simulink model "all_afc_0001_0365"  (R2026a)
settings: Solver=ode15s  StopTime=simTime  FixedStep=5e-05  RelTol=1e-06  AbsTol=1e-06
undefined symbols (not defined in the file): AF_sensor_tol, fault_time, fuel_inj_tol, MAF_sensor_tol, measureTime, simTime, spec_num
(part 3 of 3)

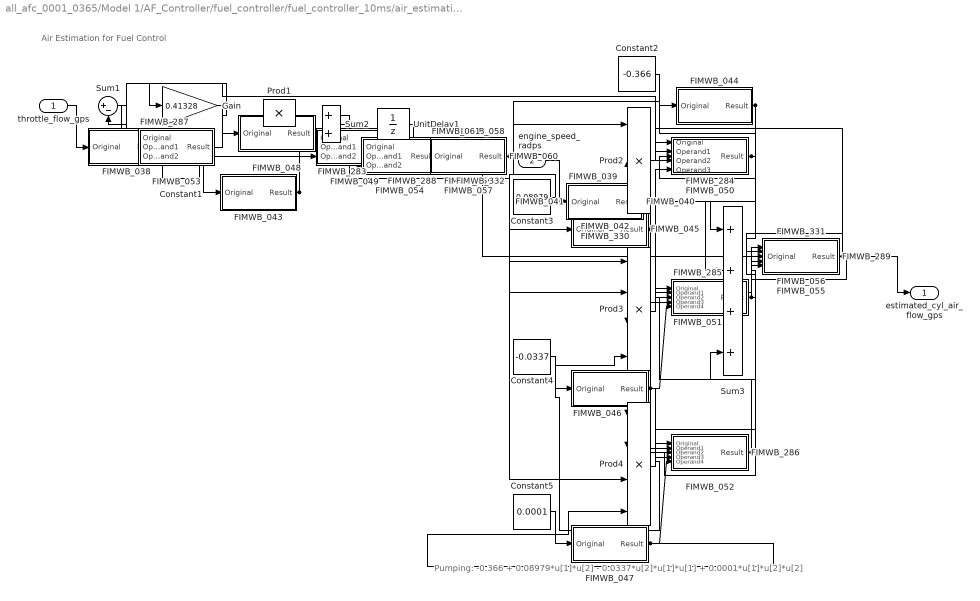
== system all_afc_0001_0365/Model 1/AF_Controller/fuel_controller/fuel_controller_10ms/air_estimation ==
  note: Air Estimation for Fuel Control
  note: Pumping: -0.366 + 0.08979*u[1]*u[2] - 0.0337*u[2]*u[1]*u[1] + 0.0001*u[1]*u[2]*u[2]
  throttle_flow_gps : Inport
  engine_speed_radps : Inport  Port=2
  Constant1 : Constant  Value=0.01  OutDataTypeStr=single  SampleTime=-1
      settings: AttributesFormatString=Sample Time (s)
  Constant2 : Constant  Value=-0.366  OutDataTypeStr=single  SampleTime=-1
  Constant3 : Constant  Value=0.08979  OutDataTypeStr=single  SampleTime=-1
  Constant4 : Constant  Value=-0.0337  OutDataTypeStr=single  SampleTime=-1
  Constant5 : Constant  Value=0.0001  OutDataTypeStr=single  SampleTime=-1
  FIMWB_038 : Subsystem  Tag=fimwb.fault.38
  FIMWB_039 : Subsystem  Tag=fimwb.fault.39
  FIMWB_040 : Subsystem  Tag=fimwb.fault.40
  FIMWB_041 : Subsystem  Tag=fimwb.fault.41
  FIMWB_042 : Subsystem  Tag=fimwb.fault.42
  FIMWB_043 : Subsystem  Tag=fimwb.fault.43
  FIMWB_044 : Subsystem  Tag=fimwb.fault.44
  FIMWB_045 : Subsystem  Tag=fimwb.fault.45
  FIMWB_046 : Subsystem  Tag=fimwb.fault.46
  FIMWB_047 : Subsystem  Tag=fimwb.fault.47
  FIMWB_048 : Subsystem  Tag=fimwb.fault.48
  FIMWB_049 : Subsystem  Tag=fimwb.fault.49
  FIMWB_050 : Subsystem  Tag=fimwb.fault.50
  FIMWB_051 : Subsystem  Tag=fimwb.fault.51
  FIMWB_052 : Subsystem  Tag=fimwb.fault.52
  FIMWB_053 : Subsystem  Tag=fimwb.fault.53
  FIMWB_054 : Subsystem  Tag=fimwb.fault.54
  FIMWB_055 : Subsystem  Tag=fimwb.fault.55
  FIMWB_056 : Subsystem  Tag=fimwb.fault.56
  FIMWB_057 : Subsystem  Tag=fimwb.fault.57
  FIMWB_058 : Subsystem  Tag=fimwb.fault.58
  FIMWB_059 : Subsystem  Tag=fimwb.fault.59
  FIMWB_060 : Subsystem  Tag=fimwb.fault.60
  FIMWB_061 : Subsystem  Tag=fimwb.fault.61
  FIMWB_283 : Subsystem  Tag=fimwb.fault.283
  FIMWB_284 : Subsystem  Tag=fimwb.fault.284
  FIMWB_285 : Subsystem  Tag=fimwb.fault.285
  FIMWB_286 : Subsystem  Tag=fimwb.fault.286
  FIMWB_287 : Subsystem  Tag=fimwb.fault.287
  FIMWB_288 : Subsystem  Tag=fimwb.fault.288
  FIMWB_289 : Subsystem  Tag=fimwb.fault.289
  FIMWB_330 : Subsystem  Tag=fimwb.fault.330
  FIMWB_331 : Subsystem  Tag=fimwb.fault.331
  FIMWB_332 : Subsystem  Tag=fimwb.fault.332
  Gain : Gain  Gain=0.41328  ParamDataTypeStr=single  OutDataTypeStr=Inherit: Inherit via back propagation  RndMeth=Simplest  SaturateOnIntegerOverflow=on
      settings: AttributesFormatString=RT/Vm
  Prod1 : Product  OutDataTypeStr=Inherit: Inherit via back propagation  RndMeth=Simplest
  Prod2 : Product  Inputs=3  OutDataTypeStr=Inherit: Inherit via back propagation  RndMeth=Simplest
  Prod3 : Product  Inputs=4  OutDataTypeStr=Inherit: Inherit via back propagation  RndMeth=Simplest
  Prod4 : Product  Inputs=4  OutDataTypeStr=Inherit: Inherit via back propagation  RndMeth=Simplest
  Sum1 : Sum  Inputs=|+-  OutDataTypeStr=Inherit: Inherit via back propagation  InputSameDT=on  RndMeth=Simplest
  Sum2 : Sum  OutDataTypeStr=Inherit: Inherit via back propagation  InputSameDT=on  RndMeth=Simplest
  Sum3 : Sum  Inputs=++++  OutDataTypeStr=Inherit: Inherit via back propagation  InputSameDT=on  RndMeth=Simplest
  UnitDelay1 : UnitDelay  InitialCondition=0.982  SampleTime=-1
      settings: AttributesFormatString=p0 = %<InitialCondition> (bar)
  estimated_cyl_air_flow_gps : Outport  VectorParamsAs1DForOutWhenUnconnected=off
  wires:
  Prod1/1 -> FIMWB_283/1(Original)
  Prod2/1 -> FIMWB_284/1(Original)
  Prod3/1 -> FIMWB_285/1(Original)
  Prod4/1 -> FIMWB_286/1(Original)
  Sum1/1 -> FIMWB_287/1(Original)
  Sum2/1 -> FIMWB_288/1(Original)
  Sum3/1 -> FIMWB_289/1(Original)
  engine_speed_radps/1 -> FIMWB_330/1(Original)
  FIMWB_330/1(Result) -> FIMWB_039/1(Original), FIMWB_040/1(Original), FIMWB_041/1(Original), FIMWB_042/1(Original)
  FIMWB_289/1(Result) -> FIMWB_331/1(Original)
  FIMWB_331/1(Result) -> FIMWB_055/1(Original), FIMWB_056/1(Original)
  UnitDelay1/1 -> FIMWB_332/1(Original)
  FIMWB_332/1(Result) -> FIMWB_057/1(Original), FIMWB_058/1(Original), FIMWB_059/1(Original), FIMWB_060/1(Original), FIMWB_061/1(Original)
  throttle_flow_gps/1 -> FIMWB_038/1(Original)
  FIMWB_038/1(Result) -> Sum1/1, FIMWB_287/2(Operand1)
  FIMWB_039/1(Result) -> Prod2/2, FIMWB_284/3(Operand2)
  FIMWB_040/1(Result) -> Prod3/3, FIMWB_285/4(Operand3)
  FIMWB_041/1(Result) -> Prod4/1, FIMWB_286/2(Operand1)
  FIMWB_042/1(Result) -> Prod4/2, FIMWB_286/3(Operand2)
  Constant1/1 -> FIMWB_043/1(Original)
  FIMWB_043/1(Result) -> Prod1/2, FIMWB_283/3(Operand2)
  Constant2/1 -> FIMWB_044/1(Original)
  FIMWB_044/1(Result) -> Sum3/1, FIMWB_289/2(Operand1)
  Constant3/1 -> FIMWB_045/1(Original)
  FIMWB_045/1(Result) -> Prod2/3, FIMWB_284/4(Operand3)
  Constant4/1 -> FIMWB_046/1(Original)
  FIMWB_046/1(Result) -> Prod3/4, FIMWB_285/5(Operand4)
  Constant5/1 -> FIMWB_047/1(Original)
  FIMWB_047/1(Result) -> Prod4/4, FIMWB_286/5(Operand4)
  Gain/1 -> FIMWB_048/1(Original)
  FIMWB_048/1(Result) -> Prod1/1, FIMWB_283/2(Operand1)
  FIMWB_283/1(Result) -> FIMWB_049/1(Original)
  FIMWB_049/1(Result) -> Sum2/1, FIMWB_288/2(Operand1)
  FIMWB_284/1(Result) -> FIMWB_050/1(Original)
  FIMWB_050/1(Result) -> Sum3/2, FIMWB_289/3(Operand2)
  FIMWB_285/1(Result) -> FIMWB_051/1(Original)
  FIMWB_051/1(Result) -> Sum3/3, FIMWB_289/4(Operand3)
  FIMWB_286/1(Result) -> FIMWB_052/1(Original)
  FIMWB_052/1(Result) -> Sum3/4, FIMWB_289/5(Operand4)
  FIMWB_287/1(Result) -> FIMWB_053/1(Original)
  FIMWB_053/1(Result) -> Gain/1
  FIMWB_288/1(Result) -> FIMWB_054/1(Original)
  FIMWB_054/1(Result) -> UnitDelay1/1
  FIMWB_055/1(Result) -> Sum1/2, FIMWB_287/3(Operand2)
  FIMWB_056/1(Result) -> estimated_cyl_air_flow_gps/1
  FIMWB_057/1(Result) -> Prod2/1, FIMWB_284/2(Operand1)
  FIMWB_058/1(Result) -> Prod3/1, FIMWB_285/2(Operand1)
  FIMWB_059/1(Result) -> Prod3/2, FIMWB_285/3(Operand2)
  FIMWB_060/1(Result) -> Prod4/3, FIMWB_286/4(Operand3)
  FIMWB_061/1(Result) -> Sum2/2, FIMWB_288/3(Operand2)

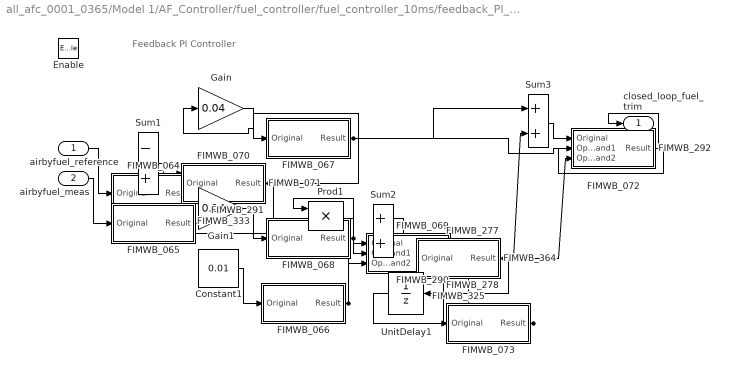
== system all_afc_0001_0365/Model 1/AF_Controller/fuel_controller/fuel_controller_10ms/feedback_PI_controller ==
  note: Feedback PI Controller
  airbyfuel_reference : Inport
  airbyfuel_meas : Inport  Port=2
  Enable : EnablePort
  Constant1 : Constant  Value=0.01  OutDataTypeStr=single  SampleTime=-1
      settings: AttributesFormatString=Sample Time [s]
  FIMWB_064 : Subsystem  Tag=fimwb.fault.64
  FIMWB_065 : Subsystem  Tag=fimwb.fault.65
  FIMWB_066 : Subsystem  Tag=fimwb.fault.66
  FIMWB_067 : Subsystem  Tag=fimwb.fault.67
  FIMWB_068 : Subsystem  Tag=fimwb.fault.68
  FIMWB_069 : Subsystem  Tag=fimwb.fault.69
  FIMWB_070 : Subsystem  Tag=fimwb.fault.70
  FIMWB_071 : Subsystem  Tag=fimwb.fault.71
  FIMWB_072 : Subsystem  Tag=fimwb.fault.72
  FIMWB_073 : Subsystem  Tag=fimwb.fault.73
  FIMWB_277 : Subsystem  Tag=fimwb.fault.277
  FIMWB_278 : Subsystem  Tag=fimwb.fault.278
  FIMWB_290 : Subsystem  Tag=fimwb.fault.290
  FIMWB_291 : Subsystem  Tag=fimwb.fault.291
  FIMWB_292 : Subsystem  Tag=fimwb.fault.292
  FIMWB_325 : Subsystem  Tag=fimwb.fault.325
  FIMWB_333 : Subsystem  Tag=fimwb.fault.333
  FIMWB_364 : Subsystem  Tag=fimwb.fault.364
  Gain : Gain  Gain=0.04  ParamDataTypeStr=single  OutDataTypeStr=Inherit: Inherit via back propagation  RndMeth=Simplest  SaturateOnIntegerOverflow=on
      settings: AttributesFormatString=Proportional Gain
  Gain1 : Gain  Gain=0.14  ParamDataTypeStr=single  OutDataTypeStr=Inherit: Inherit via back propagation  RndMeth=Simplest  SaturateOnIntegerOverflow=on
      settings: AttributesFormatString=Integral Gain
  Prod1 : Product  OutDataTypeStr=Inherit: Inherit via back propagation  RndMeth=Simplest
  Sum1 : Sum  Inputs=-+  OutDataTypeStr=Inherit: Inherit via back propagation  InputSameDT=on  RndMeth=Simplest
  Sum2 : Sum  OutDataTypeStr=Inherit: Inherit via back propagation  InputSameDT=on  RndMeth=Simplest
  Sum3 : Sum  OutDataTypeStr=Inherit: Inherit via back propagation  InputSameDT=on  RndMeth=Simplest
  UnitDelay1 : UnitDelay  SampleTime=-1
      settings: AttributesFormatString=Initial Value = 0
  closed_loop_fuel_trim : Outport  VectorParamsAs1DForOutWhenUnconnected=off
  wires:
  Prod1/1 -> FIMWB_290/1(Original)
  Sum1/1 -> FIMWB_291/1(Original)
  Sum3/1 -> FIMWB_292/1(Original)
  Sum2/1 -> FIMWB_325/1(Original)
  FIMWB_291/1(Result) -> FIMWB_333/1(Original)
  FIMWB_333/1(Result) -> FIMWB_070/1(Original), FIMWB_071/1(Original)
  FIMWB_325/1(Result) -> FIMWB_364/1(Original)
  FIMWB_364/1(Result) -> FIMWB_277/1(Original), FIMWB_278/1(Original)
  airbyfuel_reference/1 -> FIMWB_064/1(Original)
  FIMWB_064/1(Result) -> Sum1/1, FIMWB_291/2(Operand1)
  airbyfuel_meas/1 -> FIMWB_065/1(Original)
  FIMWB_065/1(Result) -> Sum1/2, FIMWB_291/3(Operand2)
  Constant1/1 -> FIMWB_066/1(Original)
  FIMWB_066/1(Result) -> Prod1/2, FIMWB_290/3(Operand2)
  Gain/1 -> FIMWB_067/1(Original)
  FIMWB_067/1(Result) -> Sum3/1, FIMWB_292/2(Operand1)
  Gain1/1 -> FIMWB_068/1(Original)
  FIMWB_068/1(Result) -> Prod1/1, FIMWB_290/2(Operand1)
  FIMWB_290/1(Result) -> FIMWB_069/1(Original)
  FIMWB_069/1(Result) -> Sum2/1, FIMWB_325/2(Operand1)
  FIMWB_070/1(Result) -> Gain/1
  FIMWB_071/1(Result) -> Gain1/1
  FIMWB_292/1(Result) -> FIMWB_072/1(Original)
  FIMWB_072/1(Result) -> closed_loop_fuel_trim/1
  UnitDelay1/1 -> FIMWB_073/1(Original)
  FIMWB_073/1(Result) -> Sum2/2, FIMWB_325/3(Operand2)
  FIMWB_277/1(Result) -> Sum3/2, FIMWB_292/3(Operand2)
  FIMWB_278/1(Result) -> UnitDelay1/1

== system all_afc_0001_0365/Model 1/AF_Controller/fuel_controller/fuel_controller_10ms/feedforward_controller ==
  note: Feedforward Controller
  estimated_cyl_air_flow_gps : Inport
  airbyfuel_reference : Inport  Port=2
  FIMWB_075 : Subsystem  Tag=fimwb.fault.75
  FIMWB_076 : Subsystem  Tag=fimwb.fault.76
  FIMWB_077 : Subsystem  Tag=fimwb.fault.77
  FIMWB_293 : Subsystem  Tag=fimwb.fault.293
  Product : Product  Inputs=*/  RndMeth=Simplest  SaturateOnIntegerOverflow=on  OutDataTypeStr=Inherit: Same as first input
  desired_fuel_mass_gps : Outport  VectorParamsAs1DForOutWhenUnconnected=off
  wires:
  Product/1 -> FIMWB_293/1(Original)
  estimated_cyl_air_flow_gps/1 -> FIMWB_075/1(Original)
  FIMWB_075/1(Result) -> Product/1, FIMWB_293/2(Operand1)
  airbyfuel_reference/1 -> FIMWB_076/1(Original)
  FIMWB_076/1(Result) -> Product/2, FIMWB_293/3(Operand2)
  FIMWB_293/1(Result) -> FIMWB_077/1(Original)
  FIMWB_077/1(Result) -> desired_fuel_mass_gps/1

== system all_afc_0001_0365/Model 1/AF_Controller/fuel_controller/fuel_controller_mode_10ms/FIMWB_079 ==
  Original : Inport
  Result : Outport
  wires:
  Original/1 -> Result/1

== system all_afc_0001_0365/Model 1/AF_Controller/fuel_controller/fuel_controller_mode_10ms/FIMWB_080 ==
  Original : Inport
  Result : Outport
  wires:
  Original/1 -> Result/1

== system all_afc_0001_0365/Model 1/AF_Controller/fuel_controller/fuel_controller_mode_10ms/FIMWB_081 ==
  Original : Inport
  Result : Outport
  wires:
  Original/1 -> Result/1

== system all_afc_0001_0365/Model 1/AF_Controller/fuel_controller/fuel_controller_mode_10ms/FIMWB_082 ==
  Original : Inport
  Result : Outport
  wires:
  Original/1 -> Result/1

== system all_afc_0001_0365/Model 1/AF_Controller/fuel_controller/fuel_controller_mode_10ms/FIMWB_083 ==
  Original : Inport
  Result : Outport
  wires:
  Original/1 -> Result/1

== system all_afc_0001_0365/Model 1/AF_Controller/fuel_controller/fuel_controller_mode_10ms/FIMWB_084 ==
  Original : Inport
  Result : Outport
  wires:
  Original/1 -> Result/1

== system all_afc_0001_0365/Model 1/AF_Controller/fuel_controller/fuel_controller_mode_10ms/FIMWB_085 ==
  Original : Inport
  Result : Outport
  wires:
  Original/1 -> Result/1

== system all_afc_0001_0365/Model 1/AF_Controller/fuel_controller/fuel_controller_mode_10ms/FIMWB_086 ==
  Original : Inport
  Result : Outport
  wires:
  Original/1 -> Result/1

== system all_afc_0001_0365/Model 1/AF_Controller/fuel_controller/fuel_controller_mode_10ms/FIMWB_087 ==
  Original : Inport
  Result : Outport
  wires:
  Original/1 -> Result/1

== system all_afc_0001_0365/Model 1/AF_Controller/fuel_controller/fuel_controller_mode_10ms/FIMWB_097 ==
  Original : Inport
  Result : Outport
  wires:
  Original/1 -> Result/1

== system all_afc_0001_0365/Model 1/AF_Controller/fuel_controller/fuel_controller_mode_10ms/FIMWB_098 ==
  Original : Inport
  Result : Outport
  wires:
  Original/1 -> Result/1

== system all_afc_0001_0365/Model 1/AF_Controller/fuel_controller/fuel_controller_mode_10ms/FIMWB_108 ==
  Original : Inport
  Result : Outport
  wires:
  Original/1 -> Result/1

== system all_afc_0001_0365/Model 1/AF_Controller/fuel_controller/fuel_controller_mode_10ms/FIMWB_268 ==
  Original : Inport
  Result : Outport
  wires:
  Original/1 -> Result/1

== system all_afc_0001_0365/Model 1/AF_Controller/fuel_controller/fuel_controller_mode_10ms/FIMWB_294 ==
  Original : Inport
  Operand1 : Inport  Port=2
  Operand2 : Inport  Port=3
  Operand3 : Inport  Port=4
  Unused2 : Terminator
  Unused3 : Terminator
  Unused4 : Terminator
  Result : Outport
  wires:
  Original/1 -> Result/1
  Operand1/1 -> Unused2/1
  Operand2/1 -> Unused3/1
  Operand3/1 -> Unused4/1

== system all_afc_0001_0365/Model 1/AF_Controller/fuel_controller/fuel_controller_mode_10ms/FIMWB_295 ==
  Original : Inport
  Operand1 : Inport  Port=2
  Unused2 : Terminator
  Result : Outport
  wires:
  Original/1 -> Result/1
  Operand1/1 -> Unused2/1

== system all_afc_0001_0365/Model 1/AF_Controller/fuel_controller/fuel_controller_mode_10ms/FIMWB_324 ==
  Original : Inport
  Operand1 : Inport  Port=2
  Operand2 : Inport  Port=3
  Unused2 : Terminator
  Unused3 : Terminator
  Result : Outport
  wires:
  Original/1 -> Result/1
  Operand1/1 -> Unused2/1
  Operand2/1 -> Unused3/1

== system all_afc_0001_0365/Model 1/AF_Controller/fuel_controller/fuel_controller_mode_10ms/FIMWB_334 ==
  Original : Inport
  Result : Outport
  wires:
  Original/1 -> Result/1

== system all_afc_0001_0365/Model 1/AF_Controller/fuel_controller/fuel_controller_mode_10ms/FIMWB_337 ==
  Original : Inport
  Result : Outport
  wires:
  Original/1 -> Result/1

== system all_afc_0001_0365/Model 1/AF_Controller/fuel_controller/fuel_controller_mode_10ms/normal_mode_detection ==
  note: Normal Mode Detection (Cold Start to Normal)
  note: NOTE: For first 10 seconds, controller uses only feedforward control to ignore the initialization issue.
  FIMWB_088 : Subsystem  Tag=fimwb.fault.88
  FIMWB_089 : Subsystem  Tag=fimwb.fault.89
  FIMWB_090 : Subsystem  Tag=fimwb.fault.90
  FIMWB_091 : Subsystem  Tag=fimwb.fault.91
  FIMWB_092 : Subsystem  Tag=fimwb.fault.92
  FIMWB_093 : Subsystem  Tag=fimwb.fault.93
  FIMWB_094 : Subsystem  Tag=fimwb.fault.94
  FIMWB_095 : Subsystem  Tag=fimwb.fault.95
  FIMWB_096 : Subsystem  Tag=fimwb.fault.96
  FIMWB_296 : Subsystem  Tag=fimwb.fault.296
  FIMWB_297 : Subsystem  Tag=fimwb.fault.297
  FIMWB_298 : Subsystem  Tag=fimwb.fault.298
  FIMWB_335 : Subsystem  Tag=fimwb.fault.335
  FIMWB_336 : Subsystem  Tag=fimwb.fault.336
  Logical Operator : Logic  Operator=OR  OutDataTypeStr=boolean
  Relational Operator : RelationalOperator  OutDataTypeStr=boolean  InputSameDT=off
  Sum : Sum
  Unit Delay1 : UnitDelay  SampleTime=-1
      settings: AttributesFormatString=Initial Value = 0
  Unit Delay2 : UnitDelay  SampleTime=-1
      settings: AttributesFormatString=Initial Value = 0
  normal_mode_start_sec : Constant  Value=10  OutDataTypeStr=single  SampleTime=-1
      settings: AttributesFormatString=Normal Mode Start Time (s)
  sampling_sec : Constant  Value=0.01  OutDataTypeStr=single  SampleTime=-1
      settings: AttributesFormatString=Sample Time (s)
  normal_on : Outport  VectorParamsAs1DForOutWhenUnconnected=off
  wires:
  Logical Operator/1 -> FIMWB_296/1(Original)
  Relational Operator/1 -> FIMWB_297/1(Original)
  Sum/1 -> FIMWB_298/1(Original)
  FIMWB_296/1(Result) -> FIMWB_335/1(Original)
  FIMWB_335/1(Result) -> FIMWB_088/1(Original), FIMWB_089/1(Original)
  FIMWB_298/1(Result) -> FIMWB_336/1(Original)
  FIMWB_336/1(Result) -> FIMWB_091/1(Original), FIMWB_092/1(Original)
  FIMWB_088/1(Result) -> Unit Delay1/1
  FIMWB_089/1(Result) -> normal_on/1
  FIMWB_297/1(Result) -> FIMWB_090/1(Original)
  FIMWB_090/1(Result) -> Logical Operator/1, FIMWB_296/2(Operand1)
  FIMWB_091/1(Result) -> Relational Operator/1, FIMWB_297/2(Operand1)
  FIMWB_092/1(Result) -> Unit Delay2/1
  Unit Delay1/1 -> FIMWB_093/1(Original)
  FIMWB_093/1(Result) -> Logical Operator/2, FIMWB_296/3(Operand2)
  Unit Delay2/1 -> FIMWB_094/1(Original)
  FIMWB_094/1(Result) -> Sum/1, FIMWB_298/2(Operand1)
  normal_mode_start_sec/1 -> FIMWB_095/1(Original)
  FIMWB_095/1(Result) -> Relational Operator/2, FIMWB_297/3(Operand2)
  sampling_sec/1 -> FIMWB_096/1(Original)
  FIMWB_096/1(Result) -> Sum/2, FIMWB_298/3(Operand2)

== system all_afc_0001_0365/Model 1/AF_Controller/fuel_controller/fuel_controller_mode_10ms/power_mode_detection ==
  note: Power Mode Detection
  throttle_angle : Inport
  Constant : Constant  Value=50  OutDataTypeStr=single
      settings: AttributesFormatString=Base
  Constant1 : Constant  Value=20  OutDataTypeStr=single
      settings: AttributesFormatString=Hysteresis
  FIMWB_099 : Subsystem  Tag=fimwb.fault.99
  FIMWB_100 : Subsystem  Tag=fimwb.fault.100
  FIMWB_101 : Subsystem  Tag=fimwb.fault.101
  FIMWB_102 : Subsystem  Tag=fimwb.fault.102
  FIMWB_103 : Subsystem  Tag=fimwb.fault.103
  FIMWB_104 : Subsystem  Tag=fimwb.fault.104
  FIMWB_105 : Subsystem  Tag=fimwb.fault.105
  FIMWB_106 : Subsystem  Tag=fimwb.fault.106
  FIMWB_107 : Subsystem  Tag=fimwb.fault.107
  FIMWB_299 : Subsystem  Tag=fimwb.fault.299
  FIMWB_300 : Subsystem  Tag=fimwb.fault.300
  FIMWB_338 : Subsystem  Tag=fimwb.fault.338
  FIMWB_339 : Subsystem  Tag=fimwb.fault.339
  Relational Operator1 : RelationalOperator  OutDataTypeStr=boolean  InputSameDT=off
  Sum : Sum
  Switch : Switch  Criteria=u2 ~= 0  SaturateOnIntegerOverflow=off  InputSameDT=off
  Unit Delay1 : UnitDelay  SampleTime=-1
      settings: AttributesFormatString=Initial Value = 0
  power_on : Outport  VectorParamsAs1DForOutWhenUnconnected=off
  wires:
  Relational Operator1/1 -> FIMWB_299/1(Original)
  Sum/1 -> FIMWB_300/1(Original)
  Constant/1 -> FIMWB_338/1(Original)
  FIMWB_338/1(Result) -> FIMWB_100/1(Original), FIMWB_101/1(Original)
  FIMWB_299/1(Result) -> FIMWB_339/1(Original)
  FIMWB_339/1(Result) -> FIMWB_103/1(Original), FIMWB_104/1(Original)
  throttle_angle/1 -> FIMWB_099/1(Original)
  FIMWB_099/1(Result) -> Relational Operator1/1, FIMWB_299/2(Operand1)
  FIMWB_100/1(Result) -> Sum/1, FIMWB_300/2(Operand1)
  FIMWB_101/1(Result) -> Switch/1
  Constant1/1 -> FIMWB_102/1(Original)
  FIMWB_102/1(Result) -> Sum/2, FIMWB_300/3(Operand2)
  FIMWB_103/1(Result) -> Unit Delay1/1
  FIMWB_104/1(Result) -> power_on/1
  FIMWB_300/1(Result) -> FIMWB_105/1(Original)
  FIMWB_105/1(Result) -> Switch/3
  Switch/1 -> FIMWB_106/1(Original)
  FIMWB_106/1(Result) -> Relational Operator1/2, FIMWB_299/3(Operand2)
  Unit Delay1/1 -> FIMWB_107/1(Original)
  FIMWB_107/1(Result) -> Switch/2

== system all_afc_0001_0365/Model 1/AF_Controller/fuel_controller/fuel_controller_mode_10ms/sensor_failure_detection ==
  note: A/F Sensor Failuer Detection
  airbyfuel_meas : Inport
  FIMWB_109 : Subsystem  Tag=fimwb.fault.109
  FIMWB_110 : Subsystem  Tag=fimwb.fault.110
  FIMWB_111 : Subsystem  Tag=fimwb.fault.111
  FIMWB_112 : Subsystem  Tag=fimwb.fault.112
  FIMWB_113 : Subsystem  Tag=fimwb.fault.113
  FIMWB_114 : Subsystem  Tag=fimwb.fault.114
  FIMWB_301 : Subsystem  Tag=fimwb.fault.301
  FIMWB_302 : Subsystem  Tag=fimwb.fault.302
  FIMWB_340 : Subsystem  Tag=fimwb.fault.340
  Logical Operator : Logic  Operator=OR  OutDataTypeStr=boolean
  Relational Operator : RelationalOperator  Operator=<=  OutDataTypeStr=boolean  InputSameDT=off
  Unit Delay : UnitDelay  SampleTime=-1
      settings: AttributesFormatString=Initial Value = 0
  threshold : Constant  Value=-1  OutDataTypeStr=single
  fail_on : Outport  VectorParamsAs1DForOutWhenUnconnected=off
  wires:
  Logical Operator/1 -> FIMWB_301/1(Original)
  Relational Operator/1 -> FIMWB_302/1(Original)
  FIMWB_301/1(Result) -> FIMWB_340/1(Original)
  FIMWB_340/1(Result) -> FIMWB_110/1(Original), FIMWB_111/1(Original)
  airbyfuel_meas/1 -> FIMWB_109/1(Original)
  FIMWB_109/1(Result) -> Relational Operator/1, FIMWB_302/2(Operand1)
  FIMWB_110/1(Result) -> Unit Delay/1
  FIMWB_111/1(Result) -> fail_on/1
  FIMWB_302/1(Result) -> FIMWB_112/1(Original)
  FIMWB_112/1(Result) -> Logical Operator/1, FIMWB_301/2(Operand1)
  Unit Delay/1 -> FIMWB_113/1(Original)
  FIMWB_113/1(Result) -> Logical Operator/2, FIMWB_301/3(Operand2)
  threshold/1 -> FIMWB_114/1(Original)
  FIMWB_114/1(Result) -> Relational Operator/2, FIMWB_302/3(Operand2)

== system all_afc_0001_0365/Model 1/AF_Controller/fuel_controller/fuel_controller_pwon/FIMWB_115 ==
  Original : Inport
  Result : Outport
  wires:
  Original/1 -> Result/1

== system all_afc_0001_0365/Model 1/AF_Controller/fuel_controller/fuel_controller_pwon/FIMWB_116 ==
  Original : Inport
  Result : Outport
  wires:
  Original/1 -> Result/1

== system all_afc_0001_0365/Model 1/AF_Controller/fuel_controller/fuel_controller_pwon/FIMWB_117 ==
  Original : Inport
  Result : Outport
  wires:
  Original/1 -> Result/1

== system all_afc_0001_0365/Model 1/AF_Controller/fuel_controller/fuel_controller_pwon/FIMWB_118 ==
  Original : Inport
  Result : Outport
  wires:
  Original/1 -> Result/1

== system all_afc_0001_0365/Model 1/Cylinder and Exhaust/A//F_sensor/Filter/FIMWB_136 ==
  Original : Inport
  Result : Outport
  wires:
  Original/1 -> Result/1

== system all_afc_0001_0365/Model 1/Cylinder and Exhaust/A//F_sensor/Filter/FIMWB_137 ==
  Original : Inport
  Result : Outport
  wires:
  Original/1 -> Result/1

== system all_afc_0001_0365/Model 1/Cylinder and Exhaust/A//F_sensor/Filter/FIMWB_138 ==
  Original : Inport
  Result : Outport
  wires:
  Original/1 -> Result/1

== system all_afc_0001_0365/Model 1/Cylinder and Exhaust/A//F_sensor/Filter/FIMWB_139 ==
  Original : Inport
  Result : Outport
  wires:
  Original/1 -> Result/1

== system all_afc_0001_0365/Model 1/Cylinder and Exhaust/A//F_sensor/Filter/FIMWB_140 ==
  Original : Inport
  Result : Outport
  wires:
  Original/1 -> Result/1

== system all_afc_0001_0365/Model 1/Cylinder and Exhaust/A//F_sensor/Filter/FIMWB_303 ==
  Original : Inport
  Operand1 : Inport  Port=2
  Operand2 : Inport  Port=3
  Unused2 : Terminator
  Unused3 : Terminator
  Result : Outport
  wires:
  Original/1 -> Result/1
  Operand1/1 -> Unused2/1
  Operand2/1 -> Unused3/1

== system all_afc_0001_0365/Model 1/Cylinder and Exhaust/A//F_sensor/Filter/FIMWB_345 ==
  Original : Inport
  Result : Outport
  wires:
  Original/1 -> Result/1

== system all_afc_0001_0365/Model 1/AF_Controller/fuel_controller/fuel_controller_10ms/air_estimation/FIMWB_038 ==
  Original : Inport
  Result : Outport
  wires:
  Original/1 -> Result/1

== system all_afc_0001_0365/Model 1/AF_Controller/fuel_controller/fuel_controller_10ms/air_estimation/FIMWB_039 ==
  Original : Inport
  Result : Outport
  wires:
  Original/1 -> Result/1

== system all_afc_0001_0365/Model 1/AF_Controller/fuel_controller/fuel_controller_10ms/air_estimation/FIMWB_040 ==
  Original : Inport
  Result : Outport
  wires:
  Original/1 -> Result/1

== system all_afc_0001_0365/Model 1/AF_Controller/fuel_controller/fuel_controller_10ms/air_estimation/FIMWB_041 ==
  Original : Inport
  Result : Outport
  wires:
  Original/1 -> Result/1

== system all_afc_0001_0365/Model 1/AF_Controller/fuel_controller/fuel_controller_10ms/air_estimation/FIMWB_042 ==
  Original : Inport
  Result : Outport
  wires:
  Original/1 -> Result/1

== system all_afc_0001_0365/Model 1/AF_Controller/fuel_controller/fuel_controller_10ms/air_estimation/FIMWB_043 ==
  Original : Inport
  Result : Outport
  wires:
  Original/1 -> Result/1

== system all_afc_0001_0365/Model 1/AF_Controller/fuel_controller/fuel_controller_10ms/air_estimation/FIMWB_044 ==
  Original : Inport
  Result : Outport
  wires:
  Original/1 -> Result/1

== system all_afc_0001_0365/Model 1/AF_Controller/fuel_controller/fuel_controller_10ms/air_estimation/FIMWB_045 ==
  Original : Inport
  Result : Outport
  wires:
  Original/1 -> Result/1

== system all_afc_0001_0365/Model 1/AF_Controller/fuel_controller/fuel_controller_10ms/air_estimation/FIMWB_046 ==
  Original : Inport
  Result : Outport
  wires:
  Original/1 -> Result/1

== system all_afc_0001_0365/Model 1/AF_Controller/fuel_controller/fuel_controller_10ms/air_estimation/FIMWB_047 ==
  Original : Inport
  Result : Outport
  wires:
  Original/1 -> Result/1

== system all_afc_0001_0365/Model 1/AF_Controller/fuel_controller/fuel_controller_10ms/air_estimation/FIMWB_048 ==
  Original : Inport
  Result : Outport
  wires:
  Original/1 -> Result/1

== system all_afc_0001_0365/Model 1/AF_Controller/fuel_controller/fuel_controller_10ms/air_estimation/FIMWB_049 ==
  Original : Inport
  Result : Outport
  wires:
  Original/1 -> Result/1

== system all_afc_0001_0365/Model 1/AF_Controller/fuel_controller/fuel_controller_10ms/air_estimation/FIMWB_050 ==
  Original : Inport
  Result : Outport
  wires:
  Original/1 -> Result/1

== system all_afc_0001_0365/Model 1/AF_Controller/fuel_controller/fuel_controller_10ms/air_estimation/FIMWB_051 ==
  Original : Inport
  Result : Outport
  wires:
  Original/1 -> Result/1

== system all_afc_0001_0365/Model 1/AF_Controller/fuel_controller/fuel_controller_10ms/air_estimation/FIMWB_052 ==
  Original : Inport
  Result : Outport
  wires:
  Original/1 -> Result/1

== system all_afc_0001_0365/Model 1/AF_Controller/fuel_controller/fuel_controller_10ms/air_estimation/FIMWB_053 ==
  Original : Inport
  Result : Outport
  wires:
  Original/1 -> Result/1

== system all_afc_0001_0365/Model 1/AF_Controller/fuel_controller/fuel_controller_10ms/air_estimation/FIMWB_054 ==
  Original : Inport
  Result : Outport
  wires:
  Original/1 -> Result/1

== system all_afc_0001_0365/Model 1/AF_Controller/fuel_controller/fuel_controller_10ms/air_estimation/FIMWB_055 ==
  Original : Inport
  Result : Outport
  wires:
  Original/1 -> Result/1

== system all_afc_0001_0365/Model 1/AF_Controller/fuel_controller/fuel_controller_10ms/air_estimation/FIMWB_056 ==
  Original : Inport
  Result : Outport
  wires:
  Original/1 -> Result/1

== system all_afc_0001_0365/Model 1/AF_Controller/fuel_controller/fuel_controller_10ms/air_estimation/FIMWB_057 ==
  Original : Inport
  Result : Outport
  wires:
  Original/1 -> Result/1

== system all_afc_0001_0365/Model 1/AF_Controller/fuel_controller/fuel_controller_10ms/air_estimation/FIMWB_058 ==
  Original : Inport
  Result : Outport
  wires:
  Original/1 -> Result/1

== system all_afc_0001_0365/Model 1/AF_Controller/fuel_controller/fuel_controller_10ms/air_estimation/FIMWB_059 ==
  Original : Inport
  Result : Outport
  wires:
  Original/1 -> Result/1

== system all_afc_0001_0365/Model 1/AF_Controller/fuel_controller/fuel_controller_10ms/air_estimation/FIMWB_060 ==
  Original : Inport
  Result : Outport
  wires:
  Original/1 -> Result/1

== system all_afc_0001_0365/Model 1/AF_Controller/fuel_controller/fuel_controller_10ms/air_estimation/FIMWB_061 ==
  Original : Inport
  Result : Outport
  wires:
  Original/1 -> Result/1

== system all_afc_0001_0365/Model 1/AF_Controller/fuel_controller/fuel_controller_10ms/air_estimation/FIMWB_283 ==
  Original : Inport
  Operand1 : Inport  Port=2
  Operand2 : Inport  Port=3
  Unused2 : Terminator
  Unused3 : Terminator
  Result : Outport
  wires:
  Original/1 -> Result/1
  Operand1/1 -> Unused2/1
  Operand2/1 -> Unused3/1

== system all_afc_0001_0365/Model 1/AF_Controller/fuel_controller/fuel_controller_10ms/air_estimation/FIMWB_284 ==
  Original : Inport
  Operand1 : Inport  Port=2
  Operand2 : Inport  Port=3
  Operand3 : Inport  Port=4
  Unused2 : Terminator
  Unused3 : Terminator
  Unused4 : Terminator
  Result : Outport
  wires:
  Original/1 -> Result/1
  Operand1/1 -> Unused2/1
  Operand2/1 -> Unused3/1
  Operand3/1 -> Unused4/1

== system all_afc_0001_0365/Model 1/AF_Controller/fuel_controller/fuel_controller_10ms/air_estimation/FIMWB_285 ==
  Original : Inport
  Operand1 : Inport  Port=2
  Operand2 : Inport  Port=3
  Operand3 : Inport  Port=4
  Operand4 : Inport  Port=5
  Unused{2..5} (4 alike) : Terminator
  Result : Outport
  wires:
  Original/1 -> Result/1
  Operand1/1 -> Unused2/1
  Operand2/1 -> Unused3/1
  Operand3/1 -> Unused4/1
  Operand4/1 -> Unused5/1

== system all_afc_0001_0365/Model 1/AF_Controller/fuel_controller/fuel_controller_10ms/air_estimation/FIMWB_286 ==
  Original : Inport
  Operand1 : Inport  Port=2
  Operand2 : Inport  Port=3
  Operand3 : Inport  Port=4
  Operand4 : Inport  Port=5
  Unused{2..5} (4 alike) : Terminator
  Result : Outport
  wires:
  Original/1 -> Result/1
  Operand1/1 -> Unused2/1
  Operand2/1 -> Unused3/1
  Operand3/1 -> Unused4/1
  Operand4/1 -> Unused5/1

== system all_afc_0001_0365/Model 1/AF_Controller/fuel_controller/fuel_controller_10ms/air_estimation/FIMWB_287 ==
  Original : Inport
  Operand1 : Inport  Port=2
  Operand2 : Inport  Port=3
  Unused2 : Terminator
  Unused3 : Terminator
  Result : Outport
  wires:
  Original/1 -> Result/1
  Operand1/1 -> Unused2/1
  Operand2/1 -> Unused3/1

== system all_afc_0001_0365/Model 1/AF_Controller/fuel_controller/fuel_controller_10ms/air_estimation/FIMWB_288 ==
  Original : Inport
  Operand1 : Inport  Port=2
  Operand2 : Inport  Port=3
  Unused2 : Terminator
  Unused3 : Terminator
  Result : Outport
  wires:
  Original/1 -> Result/1
  Operand1/1 -> Unused2/1
  Operand2/1 -> Unused3/1

== system all_afc_0001_0365/Model 1/AF_Controller/fuel_controller/fuel_controller_10ms/air_estimation/FIMWB_289 ==
  Original : Inport
  Operand1 : Inport  Port=2
  Operand2 : Inport  Port=3
  Operand3 : Inport  Port=4
  Operand4 : Inport  Port=5
  Unused{2..5} (4 alike) : Terminator
  Result : Outport
  wires:
  Original/1 -> Result/1
  Operand1/1 -> Unused2/1
  Operand2/1 -> Unused3/1
  Operand3/1 -> Unused4/1
  Operand4/1 -> Unused5/1

== system all_afc_0001_0365/Model 1/AF_Controller/fuel_controller/fuel_controller_10ms/air_estimation/FIMWB_330 ==
  Original : Inport
  Result : Outport
  wires:
  Original/1 -> Result/1

== system all_afc_0001_0365/Model 1/AF_Controller/fuel_controller/fuel_controller_10ms/air_estimation/FIMWB_331 ==
  Original : Inport
  Result : Outport
  wires:
  Original/1 -> Result/1

== system all_afc_0001_0365/Model 1/AF_Controller/fuel_controller/fuel_controller_10ms/air_estimation/FIMWB_332 ==
  Original : Inport
  Result : Outport
  wires:
  Original/1 -> Result/1

== system all_afc_0001_0365/Model 1/AF_Controller/fuel_controller/fuel_controller_10ms/feedback_PI_controller/FIMWB_064 ==
  Original : Inport
  Result : Outport
  wires:
  Original/1 -> Result/1

== system all_afc_0001_0365/Model 1/AF_Controller/fuel_controller/fuel_controller_10ms/feedback_PI_controller/FIMWB_065 ==
  Original : Inport
  Result : Outport
  wires:
  Original/1 -> Result/1

== system all_afc_0001_0365/Model 1/AF_Controller/fuel_controller/fuel_controller_10ms/feedback_PI_controller/FIMWB_066 ==
  Original : Inport
  Result : Outport
  wires:
  Original/1 -> Result/1

== system all_afc_0001_0365/Model 1/AF_Controller/fuel_controller/fuel_controller_10ms/feedback_PI_controller/FIMWB_067 ==
  Original : Inport
  Result : Outport
  wires:
  Original/1 -> Result/1

== system all_afc_0001_0365/Model 1/AF_Controller/fuel_controller/fuel_controller_10ms/feedback_PI_controller/FIMWB_068 ==
  Original : Inport
  Result : Outport
  wires:
  Original/1 -> Result/1

== system all_afc_0001_0365/Model 1/AF_Controller/fuel_controller/fuel_controller_10ms/feedback_PI_controller/FIMWB_069 ==
  Original : Inport
  Result : Outport
  wires:
  Original/1 -> Result/1

== system all_afc_0001_0365/Model 1/AF_Controller/fuel_controller/fuel_controller_10ms/feedback_PI_controller/FIMWB_070 ==
  Original : Inport
  Result : Outport
  wires:
  Original/1 -> Result/1

== system all_afc_0001_0365/Model 1/AF_Controller/fuel_controller/fuel_controller_10ms/feedback_PI_controller/FIMWB_071 ==
  Original : Inport
  Result : Outport
  wires:
  Original/1 -> Result/1

== system all_afc_0001_0365/Model 1/AF_Controller/fuel_controller/fuel_controller_10ms/feedback_PI_controller/FIMWB_072 ==
  Original : Inport
  Result : Outport
  wires:
  Original/1 -> Result/1

== system all_afc_0001_0365/Model 1/AF_Controller/fuel_controller/fuel_controller_10ms/feedback_PI_controller/FIMWB_073 ==
  Original : Inport
  Result : Outport
  wires:
  Original/1 -> Result/1

== system all_afc_0001_0365/Model 1/AF_Controller/fuel_controller/fuel_controller_10ms/feedback_PI_controller/FIMWB_277 ==
  Original : Inport
  Result : Outport
  wires:
  Original/1 -> Result/1

== system all_afc_0001_0365/Model 1/AF_Controller/fuel_controller/fuel_controller_10ms/feedback_PI_controller/FIMWB_278 ==
  Original : Inport
  Result : Outport
  wires:
  Original/1 -> Result/1

== system all_afc_0001_0365/Model 1/AF_Controller/fuel_controller/fuel_controller_10ms/feedback_PI_controller/FIMWB_290 ==
  Original : Inport
  Operand1 : Inport  Port=2
  Operand2 : Inport  Port=3
  Unused2 : Terminator
  Unused3 : Terminator
  Result : Outport
  wires:
  Original/1 -> Result/1
  Operand1/1 -> Unused2/1
  Operand2/1 -> Unused3/1

== system all_afc_0001_0365/Model 1/AF_Controller/fuel_controller/fuel_controller_10ms/feedback_PI_controller/FIMWB_291 ==
  Original : Inport
  Operand1 : Inport  Port=2
  Operand2 : Inport  Port=3
  Unused2 : Terminator
  Unused3 : Terminator
  Result : Outport
  wires:
  Original/1 -> Result/1
  Operand1/1 -> Unused2/1
  Operand2/1 -> Unused3/1

== system all_afc_0001_0365/Model 1/AF_Controller/fuel_controller/fuel_controller_10ms/feedback_PI_controller/FIMWB_292 ==
  Original : Inport
  Operand1 : Inport  Port=2
  Operand2 : Inport  Port=3
  Unused2 : Terminator
  Unused3 : Terminator
  Result : Outport
  wires:
  Original/1 -> Result/1
  Operand1/1 -> Unused2/1
  Operand2/1 -> Unused3/1

== system all_afc_0001_0365/Model 1/AF_Controller/fuel_controller/fuel_controller_10ms/feedback_PI_controller/FIMWB_325 ==
  Original : Inport
  Operand1 : Inport  Port=2
  Operand2 : Inport  Port=3
  Unused2 : Terminator
  Unused3 : Terminator
  Result : Outport
  wires:
  Original/1 -> Result/1
  Operand1/1 -> Unused2/1
  Operand2/1 -> Unused3/1

== system all_afc_0001_0365/Model 1/AF_Controller/fuel_controller/fuel_controller_10ms/feedback_PI_controller/FIMWB_333 ==
  Original : Inport
  Result : Outport
  wires:
  Original/1 -> Result/1

== system all_afc_0001_0365/Model 1/AF_Controller/fuel_controller/fuel_controller_10ms/feedback_PI_controller/FIMWB_364 ==
  Original : Inport
  Result : Outport
  wires:
  Original/1 -> Result/1

== system all_afc_0001_0365/Model 1/AF_Controller/fuel_controller/fuel_controller_10ms/feedforward_controller/FIMWB_075 ==
  Original : Inport
  Result : Outport
  wires:
  Original/1 -> Result/1

== system all_afc_0001_0365/Model 1/AF_Controller/fuel_controller/fuel_controller_10ms/feedforward_controller/FIMWB_076 ==
  Original : Inport
  Result : Outport
  wires:
  Original/1 -> Result/1

== system all_afc_0001_0365/Model 1/AF_Controller/fuel_controller/fuel_controller_10ms/feedforward_controller/FIMWB_077 ==
  Original : Inport
  Result : Outport
  wires:
  Original/1 -> Result/1

== system all_afc_0001_0365/Model 1/AF_Controller/fuel_controller/fuel_controller_10ms/feedforward_controller/FIMWB_293 ==
  Original : Inport
  Operand1 : Inport  Port=2
  Operand2 : Inport  Port=3
  Unused2 : Terminator
  Unused3 : Terminator
  Result : Outport
  wires:
  Original/1 -> Result/1
  Operand1/1 -> Unused2/1
  Operand2/1 -> Unused3/1

== system all_afc_0001_0365/Model 1/AF_Controller/fuel_controller/fuel_controller_mode_10ms/normal_mode_detection/FIMWB_088 ==
  Original : Inport
  Result : Outport
  wires:
  Original/1 -> Result/1

== system all_afc_0001_0365/Model 1/AF_Controller/fuel_controller/fuel_controller_mode_10ms/normal_mode_detection/FIMWB_089 ==
  Original : Inport
  Result : Outport
  wires:
  Original/1 -> Result/1

== system all_afc_0001_0365/Model 1/AF_Controller/fuel_controller/fuel_controller_mode_10ms/normal_mode_detection/FIMWB_090 ==
  Original : Inport
  Result : Outport
  wires:
  Original/1 -> Result/1

== system all_afc_0001_0365/Model 1/AF_Controller/fuel_controller/fuel_controller_mode_10ms/normal_mode_detection/FIMWB_091 ==
  Original : Inport
  Result : Outport
  wires:
  Original/1 -> Result/1

== system all_afc_0001_0365/Model 1/AF_Controller/fuel_controller/fuel_controller_mode_10ms/normal_mode_detection/FIMWB_092 ==
  Original : Inport
  Result : Outport
  wires:
  Original/1 -> Result/1

== system all_afc_0001_0365/Model 1/AF_Controller/fuel_controller/fuel_controller_mode_10ms/normal_mode_detection/FIMWB_093 ==
  Original : Inport
  Result : Outport
  wires:
  Original/1 -> Result/1

== system all_afc_0001_0365/Model 1/AF_Controller/fuel_controller/fuel_controller_mode_10ms/normal_mode_detection/FIMWB_094 ==
  Original : Inport
  Result : Outport
  wires:
  Original/1 -> Result/1

== system all_afc_0001_0365/Model 1/AF_Controller/fuel_controller/fuel_controller_mode_10ms/normal_mode_detection/FIMWB_095 ==
  Original : Inport
  Result : Outport
  wires:
  Original/1 -> Result/1

== system all_afc_0001_0365/Model 1/AF_Controller/fuel_controller/fuel_controller_mode_10ms/normal_mode_detection/FIMWB_096 ==
  Original : Inport
  Result : Outport
  wires:
  Original/1 -> Result/1

== system all_afc_0001_0365/Model 1/AF_Controller/fuel_controller/fuel_controller_mode_10ms/normal_mode_detection/FIMWB_296 ==
  Original : Inport
  Operand1 : Inport  Port=2
  Operand2 : Inport  Port=3
  Unused2 : Terminator
  Unused3 : Terminator
  Result : Outport
  wires:
  Original/1 -> Result/1
  Operand1/1 -> Unused2/1
  Operand2/1 -> Unused3/1

== system all_afc_0001_0365/Model 1/AF_Controller/fuel_controller/fuel_controller_mode_10ms/normal_mode_detection/FIMWB_297 ==
  Original : Inport
  Operand1 : Inport  Port=2
  Operand2 : Inport  Port=3
  Unused2 : Terminator
  Unused3 : Terminator
  Result : Outport
  wires:
  Original/1 -> Result/1
  Operand1/1 -> Unused2/1
  Operand2/1 -> Unused3/1

== system all_afc_0001_0365/Model 1/AF_Controller/fuel_controller/fuel_controller_mode_10ms/normal_mode_detection/FIMWB_298 ==
  Original : Inport
  Operand1 : Inport  Port=2
  Operand2 : Inport  Port=3
  Unused2 : Terminator
  Unused3 : Terminator
  Result : Outport
  wires:
  Original/1 -> Result/1
  Operand1/1 -> Unused2/1
  Operand2/1 -> Unused3/1

== system all_afc_0001_0365/Model 1/AF_Controller/fuel_controller/fuel_controller_mode_10ms/normal_mode_detection/FIMWB_335 ==
  Original : Inport
  Result : Outport
  wires:
  Original/1 -> Result/1

== system all_afc_0001_0365/Model 1/AF_Controller/fuel_controller/fuel_controller_mode_10ms/normal_mode_detection/FIMWB_336 ==
  Original : Inport
  Result : Outport
  wires:
  Original/1 -> Result/1

== system all_afc_0001_0365/Model 1/AF_Controller/fuel_controller/fuel_controller_mode_10ms/power_mode_detection/FIMWB_099 ==
  Original : Inport
  Result : Outport
  wires:
  Original/1 -> Result/1

== system all_afc_0001_0365/Model 1/AF_Controller/fuel_controller/fuel_controller_mode_10ms/power_mode_detection/FIMWB_100 ==
  Original : Inport
  Result : Outport
  wires:
  Original/1 -> Result/1

== system all_afc_0001_0365/Model 1/AF_Controller/fuel_controller/fuel_controller_mode_10ms/power_mode_detection/FIMWB_101 ==
  Original : Inport
  Result : Outport
  wires:
  Original/1 -> Result/1

== system all_afc_0001_0365/Model 1/AF_Controller/fuel_controller/fuel_controller_mode_10ms/power_mode_detection/FIMWB_102 ==
  Original : Inport
  Result : Outport
  wires:
  Original/1 -> Result/1

== system all_afc_0001_0365/Model 1/AF_Controller/fuel_controller/fuel_controller_mode_10ms/power_mode_detection/FIMWB_103 ==
  Original : Inport
  Result : Outport
  wires:
  Original/1 -> Result/1

== system all_afc_0001_0365/Model 1/AF_Controller/fuel_controller/fuel_controller_mode_10ms/power_mode_detection/FIMWB_104 ==
  Original : Inport
  Result : Outport
  wires:
  Original/1 -> Result/1

== system all_afc_0001_0365/Model 1/AF_Controller/fuel_controller/fuel_controller_mode_10ms/power_mode_detection/FIMWB_105 ==
  Original : Inport
  Result : Outport
  wires:
  Original/1 -> Result/1

== system all_afc_0001_0365/Model 1/AF_Controller/fuel_controller/fuel_controller_mode_10ms/power_mode_detection/FIMWB_106 ==
  Original : Inport
  Result : Outport
  wires:
  Original/1 -> Result/1

== system all_afc_0001_0365/Model 1/AF_Controller/fuel_controller/fuel_controller_mode_10ms/power_mode_detection/FIMWB_107 ==
  Original : Inport
  Result : Outport
  wires:
  Original/1 -> Result/1

== system all_afc_0001_0365/Model 1/AF_Controller/fuel_controller/fuel_controller_mode_10ms/power_mode_detection/FIMWB_299 ==
  Original : Inport
  Operand1 : Inport  Port=2
  Operand2 : Inport  Port=3
  Unused2 : Terminator
  Unused3 : Terminator
  Result : Outport
  wires:
  Original/1 -> Result/1
  Operand1/1 -> Unused2/1
  Operand2/1 -> Unused3/1

== system all_afc_0001_0365/Model 1/AF_Controller/fuel_controller/fuel_controller_mode_10ms/power_mode_detection/FIMWB_300 ==
  Original : Inport
  Operand1 : Inport  Port=2
  Operand2 : Inport  Port=3
  Unused2 : Terminator
  Unused3 : Terminator
  Result : Outport
  wires:
  Original/1 -> Result/1
  Operand1/1 -> Unused2/1
  Operand2/1 -> Unused3/1

== system all_afc_0001_0365/Model 1/AF_Controller/fuel_controller/fuel_controller_mode_10ms/power_mode_detection/FIMWB_338 ==
  Original : Inport
  Result : Outport
  wires:
  Original/1 -> Result/1

== system all_afc_0001_0365/Model 1/AF_Controller/fuel_controller/fuel_controller_mode_10ms/power_mode_detection/FIMWB_339 ==
  Original : Inport
  Result : Outport
  wires:
  Original/1 -> Result/1

== system all_afc_0001_0365/Model 1/AF_Controller/fuel_controller/fuel_controller_mode_10ms/sensor_failure_detection/FIMWB_109 ==
  Original : Inport
  Result : Outport
  wires:
  Original/1 -> Result/1

== system all_afc_0001_0365/Model 1/AF_Controller/fuel_controller/fuel_controller_mode_10ms/sensor_failure_detection/FIMWB_110 ==
  Original : Inport
  Result : Outport
  wires:
  Original/1 -> Result/1

== system all_afc_0001_0365/Model 1/AF_Controller/fuel_controller/fuel_controller_mode_10ms/sensor_failure_detection/FIMWB_111 ==
  Original : Inport
  Result : Outport
  wires:
  Original/1 -> Result/1

== system all_afc_0001_0365/Model 1/AF_Controller/fuel_controller/fuel_controller_mode_10ms/sensor_failure_detection/FIMWB_112 ==
  Original : Inport
  Result : Outport
  wires:
  Original/1 -> Result/1

== system all_afc_0001_0365/Model 1/AF_Controller/fuel_controller/fuel_controller_mode_10ms/sensor_failure_detection/FIMWB_113 ==
  Original : Inport
  Result : Outport
  wires:
  Original/1 -> Result/1

== system all_afc_0001_0365/Model 1/AF_Controller/fuel_controller/fuel_controller_mode_10ms/sensor_failure_detection/FIMWB_114 ==
  Original : Inport
  Result : Outport
  wires:
  Original/1 -> Result/1

== system all_afc_0001_0365/Model 1/AF_Controller/fuel_controller/fuel_controller_mode_10ms/sensor_failure_detection/FIMWB_301 ==
  Original : Inport
  Operand1 : Inport  Port=2
  Operand2 : Inport  Port=3
  Unused2 : Terminator
  Unused3 : Terminator
  Result : Outport
  wires:
  Original/1 -> Result/1
  Operand1/1 -> Unused2/1
  Operand2/1 -> Unused3/1

== system all_afc_0001_0365/Model 1/AF_Controller/fuel_controller/fuel_controller_mode_10ms/sensor_failure_detection/FIMWB_302 ==
  Original : Inport
  Operand1 : Inport  Port=2
  Operand2 : Inport  Port=3
  Unused2 : Terminator
  Unused3 : Terminator
  Result : Outport
  wires:
  Original/1 -> Result/1
  Operand1/1 -> Unused2/1
  Operand2/1 -> Unused3/1

== system all_afc_0001_0365/Model 1/AF_Controller/fuel_controller/fuel_controller_mode_10ms/sensor_failure_detection/FIMWB_340 ==
  Original : Inport
  Result : Outport
  wires:
  Original/1 -> Result/1
